simulink model "SLX_HoqueSimulink"  (R2025a)
settings: Solver=VariableStepAuto  StartTime=0.0  StopTime=inf  RelTol=1e-3
values from neighbouring files (symbols this model uses):
  Cd = 0.5    [SLX_HoqueMatlab.m]
  centreOfMassHeight = 0.5    [SLX_HoqueMatlab.m]
  frontExposedArea = 0.3    [SLX_HoqueMatlab.m]
  g = 9.81    [SLX_HoqueMatlab.m]
  inertia = 1    [SLX_HoqueMatlab.m]
  mass = 200    [SLX_HoqueMatlab.m]
  radius = 0.3    [SLX_HoqueMatlab.m]
  rhoAir = 1.225    [SLX_HoqueMatlab.m]
  wheelbase = 1.4    [SLX_HoqueMatlab.m]
libraries: slpidlib x2
settings Model: PacingRate=0.710000  Creator=rafiu  LastModifiedBy=rafiu

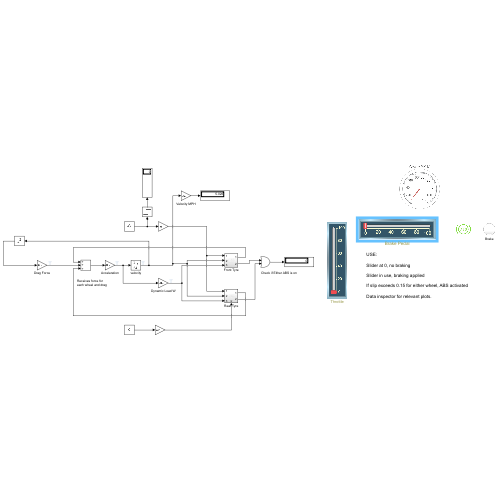
[thumbnail: Simulink's stored preview of the top-level diagram]
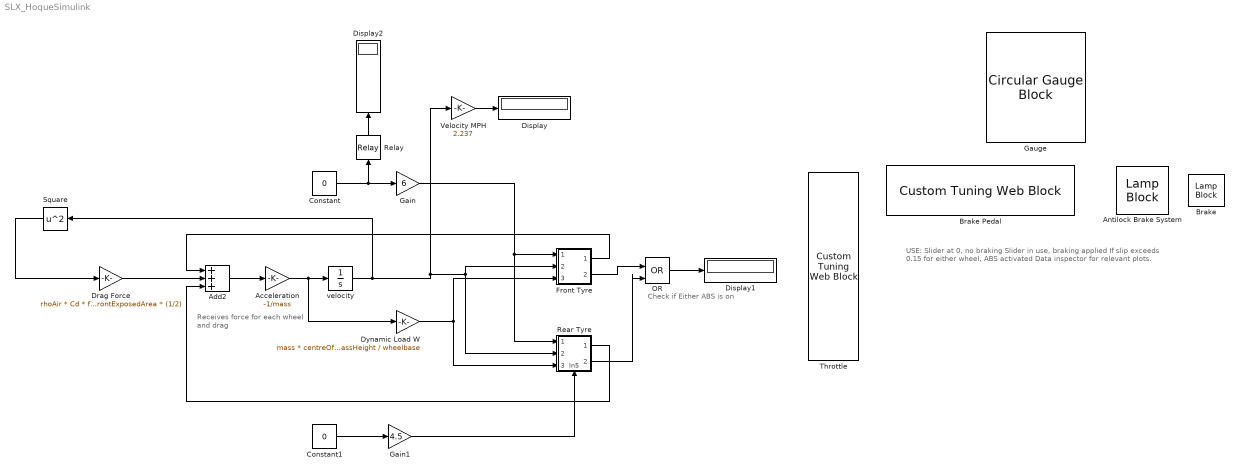
== system SLX_HoqueSimulink ==
  note: Receives force for each wheel and drag
  note: Check if Either ABS is on
  note: USE:
      |
      | Slider at 0, no braking
      |
      | Slider in use, braking applied
      |
      | If slip exceeds 0.15 for either wheel, ABS activated
      |
      | Data inspector for relevant plots.
  Acceleration : Gain  Gain=-1/mass
  Add2 : Sum  Inputs=+++
  Antilock Brake System : LampBlock  LabelPosition=Hide  DefaultColor=[192.0, 192.0, 192.0]  Icon=AntilockBrakeSystem
  Brake : LampBlock  LabelPosition=Hide  DefaultColor=[192.0, 192.0, 192.0]
  Brake Pedal : CustomTuningWebBlock  LabelPosition=Hide  ShowInitialText=on  Configuration="{\"components\":[{\"name\":\"LinearScaleComponent\",\"settings\":{\"bounds\":{\"max\":100,\"min\":0,\"tickInterval\":\"auto\"},\"internalTickHeightScaleFactor\":0.5,\"labelColor\":[255,255,200],\"labelFont\":{\"font\":\"Arial\",\"fontSize\":12},\"labelOffset\":0.05,\"labelTransparency\":1,\"needleImage\":{\"size\":[596,842],\"src\":\"data:image\\/svg+xml;base64,PD94bWwgdmVyc2lvbj0iMS4wIiBlbmNvZGluZz0idXRmLTgiPz4NCjwhLS0gR2VuZXJhdG9yOiBBZG9iZSBJbGx1c3RyYXRvciAyNS4wLjAsIFNWRyBFeHBvcnQgUGx1Zy1JbiAuIFNWRyBWZXJzaW9uOiA2LjAwIEJ1aWxkIDApICAtLT4NCjxzdmcgdmVyc2lvbj0iMS4xIg0KCSBpZD0ic3ZnOCIgeG1sbnM6Y2M9Imh0dHA6Ly9jcmVhdGl2ZWNvbW1vbnMub3JnL25zIyIgeG1sbnM6ZGM9Imh0dHA6Ly9wdXJsLm9yZy9kYy9lbGVtZW50cy8xLjEvIiB4bWxuczppbmtzY2FwZT0iaHR0cDovL3d3dy5pbmtzY2FwZS5vcmcvbmFtZXNw ...(+2420 chars)\",\"srcOrientation\":\"Right\"},\"needleOffset\":[-0.8044596912521441,-0.0642123287671233],\"needleSize\":{\"height\":0.4337797619047619,\"width\":0.07668067226890757},\"position\":[0.2829861111111111,0.04398634453781513,0.9196428571428571,0.6088789682539683],\"referencePoint\":\"auto\",\"scaleColors\":[],\"scaleColorsSize\":0.2,\"scaleDirection\":\"LR\",\"showLabels\":1,\"showMinorTicks\":0,\"showSpanLine\":1,\"showTicks\":1,\"tickColor\":[252,252,197],\"tickTransparency\":1,\"valueBarColor\":[0,114,189],\"valueBarOffset\":-0.27,\"valueBarSize\":0.1,\"valueBarTransparency\":1}},{\"name\":\"BackgroundImageComponent\",\"settings\":{\"image\":{\"size\":[380,101],\"src\":\"data:image\\/svg+xml;base64,PHN2ZyB4bWxucz0iaHR0cDovL3d3dy53My5vcmcvMjAwMC9zdmciIHhtbG5zOnhsaW5rPSJodHRwOi8vd3d3LnczLm9yZy8xOTk5L3hsaW5rIiB2aWV3Qm94PSIwIDAgMzgwIDEwMSI+PGRlZnM+PHN0eWxlPi5jbHMtMXtmaWxsOiMwMDJiNDI7fS5jbHMtMntmaWxsOiM0MjcwODI7fS5jbHMtM3tmaWxsOnVybCgjcmFkaWFsLWdyYWRpZW50KTt9LmNscy00e2ZpbGw6I2M4YzhjODtzdHJva2U6IzAwMDt9PC9zdHlsZT48cmFkaWFsR3JhZGllbnQgaWQ9InJhZGlhbC1ncmFkaWVudCIgY3g9IjE5MCIgY3k9IjUwLjUiIHI9IjI2OS4yMSIgZ3JhZGllbnRVbml0cz0idXNlclNwYWNlT25Vc2UiPjxzdG9wIG9mZnNldD0iMC4wMSIgc3RvcC1jb2xvcj0iIzNlNGY1OCIvPjxzdG9wIG9mZnNldD0iMC4wNiIgc3RvcC1jb2xvcj0iIzQ0NTc2MSIvPjxzdG9wIG9mZnNldD0iMC4xNSIgc3RvcC1jb2xvcj0iIzU1NmE3NiIvPjxzdG9wIG9mZnNldD0iMC4yNSIgc3RvcC1jb2xvcj0iIzZkODg5NSIvPjxzdG9wIG9mZnNldD0iMC4zOCIgc3RvcC1jb2xvcj0iIzhmYjJjMyIvPjxzdG9wIG9mZnNldD0iMC41MiIgc3RvcC1jb2xvcj0iI2I2ZTRmYSIvPjxzdG9wIG9mZnNldD0iMSIgc3RvcC1jb2xvcj0iIzE1NDY1NyIvPjwvcmFkaWFsR3JhZGllbnQ+PC9kZWZzPjxnIGlkPSJmcmFtZSI+PGcgaWQ9IkxheWVyXzIiIGRhdGEtbmFtZT0iTGF5ZXIgMiI+PGcgaWQ9IkxheWVyXzEtMiIgZGF0YS1uYW1lPSJMYXllciAxLTIiPjxyZWN0IGlkPSJyZWN0MTAzNiIgY2xhc3M9ImNscy0xIiB4PSIxMSIgeT0iMTEiIHdpZHRoPSIzNTgiIGhlaWdodD0iNzkiLz48cGF0aCBpZD0icGF0aDEwMzgiIGNsYXNzPSJjbHMtMiIgZD0iTTgsOFY5M0gzNzJWOFpNMzY5LDkwSDExVjExSDM2OVoiLz48cGF0aCBpZD0icGF0aDEwNDAiIGNsYXNzPSJjbHMtMyIgZD0iTTAsMFYxMDFIMzgwVjBaTTM3Miw5M0g4VjhIMzcyWiIvPjwvZz48L2c+PC9nPjxnIGlkPSJ0cmFjayI+PHBhdGggaWQ9InJlY3QxNjExIiBjbGFzcz0iY2xzLTQiIGQ9Ik0zMy4zNywyNi41OUgzNDYuNjNjNCwwLDcuMjUsMi42LDcuMjUsNS44MWgwYzAsMy4yMS0zLjI1LDUuODItNy4yNSw1LjgySDMzLjM3Yy00LDAtNy4yNS0yLjYxLTcuMjUtNS44MmgwQzI2LjEyLDI5LjE5LDI5LjM3LDI2LjU5LDMzLjM3LDI2LjU5WiIvPjwvZz48L3N2Zz4=\",\"srcOrientation\":\"horizontal\"},\"position\":[0,0,1,1],\"scaleMode\":\"0\"}},{\"name\":\"ForegroundImageComponent\",\"settings\":{\"image\":{\"size\":[0,0],\"src\":\"default\",\"srcOrientation\":[]},\"isForeground\":1,\"position\":[0,0,1,1],\"scaleMode\":\"0\"}}],\"derived\":{\"blockParameters\":{\"ForegroundColor\":[0.9882352941176471,0.9882352941176471,0.7725490196078432],\"Limits\":{\"Max\":100,\"Min\":0,\"Ticks\":\"auto\"},\"ScaleColors\":[],\"ScaleDirection\":\"Clockwise\",\"ScaleMax\":100,\"ScaleMin\":0,\"TickInterval\":\"auto\",\"fixedAspectRatio\":\"on\"}},\"settings\":{\"BindingType\":\"param\",\"aspectRatio\":3.7777777777777777,\"backgroundColor\":[0,0,0,\"1\"],\"backgroundOffset\":0,\"backgroundOpacity\":1,\"fixedAspectRatio\":\"on\",\"foregroundColor\":[252,252,196],\"orientation\":\"horizontal\",\"showBackgroundColor\":false,\"value\":0,\"version\":\"R2023a\"},\"type\":\"LinearGauge\"}"
  Constant : Constant  Value=0
  Constant1 : Constant  Value=0
  Display : Display
  Display1 : Display
  Display2 : Display
  Drag Force : Gain  Gain=rhoAir * Cd * frontExposedArea * (1/2)
  Dynamic Load W : Gain  Gain=mass * centreOfMassHeight / wheelbase
  Front Tyre : Subsystem
  Gain : Gain  Gain=6
  Gain1 : Gain  Gain=4.5
  Gauge : CircularGaugeBlock  ScaleMax=180  FontColor=[0.0, 0.0, 0.0]
  OR : Logic  Operator=OR  IconShape=distinctive  AllPortsSameDT=off  OutDataTypeStr=boolean
  Rear Tyre : Subsystem
      settings: PortSchema="{\"entries\":[{\"content\":{\"sides\":[{\"content\":{\"connectorIds\":[\"In1\",\"In2\",\"In3\"]},\"type\":\"ConnectorPlacement.EquallySpacedRectSide\",\"uuid\":\"1266f35d-f5b4-4b9c-be11-d6befbdb1413\"},{\"content\":{\"connectorIds\":[\"Out1\",\"Out2\"],\"side\":\"RIGHT\"},\"type\":\"ConnectorPlacement.EquallySpacedRectSide\",\"uuid\":\"caeb7587-b63b-4911-94e2-b6cf9e0b40d6\"},{\"content\":{\"side\":\"TOP\"},\"type\":\"ConnectorPlacement.EquallySpacedRectSide\",\"uuid\":\"79f45d0a-d588-4f96-966e-94542620e09c\"},{\"content\":{\"connectorIds\":[\"In4\"],\"side\":\"BOTTOM\"},\"type\":\"ConnectorPlacement.EquallySpacedRectSide\",\"uuid\":\"f75c0003-57c9-4cd0-88eb-cf91023de0b2\"}]},\"type\":\"ConnectorPlacement.EquallySpacedConnector\",\"uuid\":\"6a6eede2-c9ff-4d9d-a3d1-7dc9cb2ac1d3\"}],\"packageUris\":[\"http://schema.mathworks.com/mf0/Connector/R2020b\"],\"version\":\"1.0\"}"
  Relay : Relay  OnSwitchValue=0.1  OffSwitchValue=0
  Square : Math  Operator=square
  Throttle : CustomTuningWebBlock  LabelPosition=Hide  ShowInitialText=on  Configuration="{\"components\":[{\"name\":\"LinearScaleComponent\",\"settings\":{\"bounds\":{\"max\":100,\"min\":0,\"tickInterval\":\"auto\"},\"internalTickHeightScaleFactor\":0.5,\"labelColor\":[255,255,200],\"labelFont\":{\"font\":\"Arial\",\"fontSize\":12},\"labelOffset\":0.05,\"labelTransparency\":1,\"needleImage\":{\"size\":[596,842],\"src\":\"data:image\\/svg+xml;base64,PD94bWwgdmVyc2lvbj0iMS4wIiBlbmNvZGluZz0idXRmLTgiPz4NCjwhLS0gR2VuZXJhdG9yOiBBZG9iZSBJbGx1c3RyYXRvciAyNS4wLjAsIFNWRyBFeHBvcnQgUGx1Zy1JbiAuIFNWRyBWZXJzaW9uOiA2LjAwIEJ1aWxkIDApICAtLT4NCjxzdmcgdmVyc2lvbj0iMS4xIg0KCSBpZD0ic3ZnOCIgeG1sbnM6Y2M9Imh0dHA6Ly9jcmVhdGl2ZWNvbW1vbnMub3JnL25zIyIgeG1sbnM6ZGM9Imh0dHA6Ly9wdXJsLm9yZy9kYy9lbGVtZW50cy8xLjEvIiB4bWxuczppbmtzY2FwZT0iaHR0cDovL3d3dy5pbmtzY2FwZS5vcmcvbmFtZXNw ...(+2420 chars)\",\"srcOrientation\":\"horizontal\"},\"needleOffset\":[0.0642123287671233,-0.8044596912521441],\"needleSize\":{\"height\":0.07668067226890757,\"width\":0.4337797619047619},\"position\":[0.03623949579831933,0.2829861111111111,0.6088789682539683,0.9196428571428571],\"referencePoint\":\"auto\",\"scaleColors\":[],\"scaleColorsSize\":0.2,\"scaleDirection\":\"BT\",\"showLabels\":1,\"showMinorTicks\":0,\"showSpanLine\":1,\"showTicks\":1,\"tickColor\":[252,252,197],\"tickTransparency\":1,\"valueBarColor\":[0,114,189],\"valueBarOffset\":-0.27,\"valueBarSize\":0.1,\"valueBarTransparency\":1}},{\"name\":\"BackgroundImageComponent\",\"settings\":{\"image\":{\"size\":[380,101],\"src\":\"data:image\\/svg+xml;base64,PHN2ZyB4bWxucz0iaHR0cDovL3d3dy53My5vcmcvMjAwMC9zdmciIHhtbG5zOnhsaW5rPSJodHRwOi8vd3d3LnczLm9yZy8xOTk5L3hsaW5rIiB2aWV3Qm94PSIwIDAgMzgwIDEwMSI+PGRlZnM+PHN0eWxlPi5jbHMtMXtmaWxsOiMwMDJiNDI7fS5jbHMtMntmaWxsOiM0MjcwODI7fS5jbHMtM3tmaWxsOnVybCgjcmFkaWFsLWdyYWRpZW50KTt9LmNscy00e2ZpbGw6I2M4YzhjODtzdHJva2U6IzAwMDt9PC9zdHlsZT48cmFkaWFsR3JhZGllbnQgaWQ9InJhZGlhbC1ncmFkaWVudCIgY3g9IjE5MCIgY3k9IjUwLjUiIHI9IjI2OS4yMSIgZ3JhZGllbnRVbml0cz0idXNlclNwYWNlT25Vc2UiPjxzdG9wIG9mZnNldD0iMC4wMSIgc3RvcC1jb2xvcj0iIzNlNGY1OCIvPjxzdG9wIG9mZnNldD0iMC4wNiIgc3RvcC1jb2xvcj0iIzQ0NTc2MSIvPjxzdG9wIG9mZnNldD0iMC4xNSIgc3RvcC1jb2xvcj0iIzU1NmE3NiIvPjxzdG9wIG9mZnNldD0iMC4yNSIgc3RvcC1jb2xvcj0iIzZkODg5NSIvPjxzdG9wIG9mZnNldD0iMC4zOCIgc3RvcC1jb2xvcj0iIzhmYjJjMyIvPjxzdG9wIG9mZnNldD0iMC41MiIgc3RvcC1jb2xvcj0iI2I2ZTRmYSIvPjxzdG9wIG9mZnNldD0iMSIgc3RvcC1jb2xvcj0iIzE1NDY1NyIvPjwvcmFkaWFsR3JhZGllbnQ+PC9kZWZzPjxnIGlkPSJmcmFtZSI+PGcgaWQ9IkxheWVyXzIiIGRhdGEtbmFtZT0iTGF5ZXIgMiI+PGcgaWQ9IkxheWVyXzEtMiIgZGF0YS1uYW1lPSJMYXllciAxLTIiPjxyZWN0IGlkPSJyZWN0MTAzNiIgY2xhc3M9ImNscy0xIiB4PSIxMSIgeT0iMTEiIHdpZHRoPSIzNTgiIGhlaWdodD0iNzkiLz48cGF0aCBpZD0icGF0aDEwMzgiIGNsYXNzPSJjbHMtMiIgZD0iTTgsOFY5M0gzNzJWOFpNMzY5LDkwSDExVjExSDM2OVoiLz48cGF0aCBpZD0icGF0aDEwNDAiIGNsYXNzPSJjbHMtMyIgZD0iTTAsMFYxMDFIMzgwVjBaTTM3Miw5M0g4VjhIMzcyWiIvPjwvZz48L2c+PC9nPjxnIGlkPSJ0cmFjayI+PHBhdGggaWQ9InJlY3QxNjExIiBjbGFzcz0iY2xzLTQiIGQ9Ik0zMy4zNywyNi41OUgzNDYuNjNjNCwwLDcuMjUsMi42LDcuMjUsNS44MWgwYzAsMy4yMS0zLjI1LDUuODItNy4yNSw1LjgySDMzLjM3Yy00LDAtNy4yNS0yLjYxLTcuMjUtNS44MmgwQzI2LjEyLDI5LjE5LDI5LjM3LDI2LjU5LDMzLjM3LDI2LjU5WiIvPjwvZz48L3N2Zz4=\",\"srcOrientation\":\"horizontal\"},\"position\":[0,0,1,1],\"scaleMode\":\"0\"}},{\"name\":\"ForegroundImageComponent\",\"settings\":{\"image\":{\"size\":[0,0],\"src\":\"default\",\"srcOrientation\":[]},\"isForeground\":1,\"position\":[0,0,1,1],\"scaleMode\":\"0\"}}],\"derived\":{\"blockParameters\":{\"ForegroundColor\":[0.9882352941176471,0.9882352941176471,0.7725490196078432],\"Limits\":{\"Max\":100,\"Min\":0,\"Ticks\":\"auto\"},\"ScaleColors\":[],\"ScaleDirection\":\"Clockwise\",\"ScaleMax\":100,\"ScaleMin\":0,\"TickInterval\":\"auto\",\"fixedAspectRatio\":\"on\"}},\"settings\":{\"BindingType\":\"param\",\"aspectRatio\":3.7777777777777777,\"backgroundColor\":[0,0,0,\"1\"],\"backgroundOffset\":0,\"backgroundOpacity\":1,\"fixedAspectRatio\":\"on\",\"foregroundColor\":[252,252,196],\"orientation\":\"vertical\",\"showBackgroundColor\":false,\"value\":0,\"version\":\"R2023a\"},\"type\":\"LinearGauge\"}"
  Velocity MPH : Gain  Gain=2.237
  velocity : Integrator  InitialCondition=25  LimitOutput=on  LowerSaturationLimit=0.1
  wires:
  Acceleration/1 -> Dynamic Load W/1, velocity/1
  Add2/1 -> Acceleration/1
  Dynamic Load W/1 -> Rear Tyre/3(In2), Front Tyre/3(In2)
  Front Tyre/1(Out1) -> Add2/1
  Constant/1 -> Gain/1, Relay/1
  Gain/1 -> Front Tyre/1(1), Rear Tyre/1(In3)
  Velocity MPH/1 -> Display/1
  OR/1 -> Display1/1
  Front Tyre/2(Out2) -> OR/1
  Rear Tyre/2(Out2) -> OR/2
  Relay/1 -> Display2/1
  Constant1/1 -> Gain1/1
  Gain1/1 -> Rear Tyre/4(In5)
  velocity/1 -> Square/1, Velocity MPH/1, Front Tyre/2(In1), Rear Tyre/2(In1)
  Rear Tyre/1(Out1) -> Add2/3
  Square/1 -> Drag Force/1
  Drag Force/1 -> Add2/2

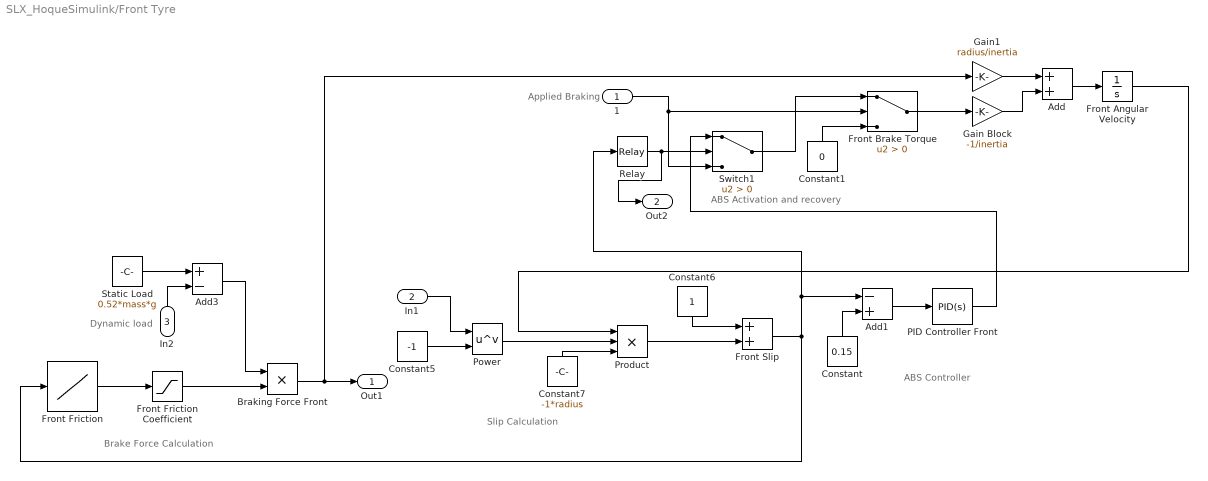
== system SLX_HoqueSimulink/Front Tyre ==
  note: Dynamic load
  note: Brake Force Calculation
  note: ABS Activation and recovery
  note: Applied Braking
  note: Slip Calculation
  note: ABS Controller
  1 : Inport
  In1 : Inport  Port=2
  In2 : Inport  Port=3
  Add : Sum
  Add1 : Sum  Inputs=-+
  Add3 : Sum  Inputs=+-
  Braking Force Front : Product
  Constant : Constant  Value=0.15
  Constant1 : Constant  Value=0
  Constant5 : Constant  Value=-1
  Constant6 : Constant
  Constant7 : Constant  Value=-1*radius
  "Front Angular Velocity " : Integrator  InitialCondition=83.33  LimitOutput=on  LowerSaturationLimit=0
  Front Brake Torque : Switch  Criteria=u2 > Threshold  SaturateOnIntegerOverflow=off  InputSameDT=off
  Front Friction : Lookup_n-D  NumberOfTableDimensions=1  BreakpointsForDimension1=[-1;-0.5;-0.29999999999999999;-0.20000000000000001;-0.14999999999999999;-0.10000000000000001;-0.050000000000000003;0;0.050000000000000003;0.10000000000000001;0.14999999999999999;0.20000000000000001;0.29999999999999999;0.5;1]  Table=[-0.10000000000000001;-0.40000000000000002;-0.75;-0.94999999999999996;-1;-0.90000000000000002;-0.59999999999999998;0;0.59999999999999998;0.90000000000000002;1;0.94999999999999996;0.75;0.40000000000000002;0.10000000000000001]  InternalRulePriority=Speed  RndMeth=Simplest
  Front Friction Coefficient : Saturate  UpperLimit=1  LowerLimit=-1
  Front Slip : Sum
  Gain Block : Gain  Gain=-1/inertia
  Gain1 : Gain  Gain=radius/inertia
  PID Controller Front : slpidlib/PID Controller  Controller=PID  Form=Parallel  TimeDomain=Continuous-time  UseExternalTs=off  SampleTime=-1  IntegratorMethod=Forward Euler  FilterMethod=Forward Euler  ControllerParametersSource=internal  P=6397.12321645697  I=564779.033744015  UseKiTs=off  D=-9.50321064069282  UseExternalDerivativeSource=off  N=94.2884376417399  UseFilter=on  TunerSelectOption=Transfer Function Based (PID Tuner App)  InitialConditionSource=internal  InitialConditionForIntegrator=0  InitialConditionForFilter=0  DifferentiatorICPrevScaledInput=0  ExternalReset=none  TrackingMode=off  Kt=1  LimitOutput=on  SatLimitsSource=internal  UpperSaturationLimit=600  LowerSaturationLimit=0  LinearizeAsGain=on  AntiWindupMode=back-calculation  Kb=1  LimitIntegrator=on  UpperIntegratorSaturationLimit=1000  LowerIntegratorSaturationLimit=-inf  POutMin=[]  POutMax=[]  IOutMin=[]  IOutMax=[]  DOutMin=[]  DOutMax=[]  NOutMin=[]  NOutMax=[]  SumOutMin=[]  SumOutMax=[]  SaturationOutMin=[]  SaturationOutMax=[]  PParamMin=[]  PParamMax=[]  IParamMin=[]  IParamMax=[]  DParamMin=[]  DParamMax=[]  NParamMin=[]  NParamMax=[]  KbParamMin=[]  KbParamMax=[]  KtParamMin=[]  KtParamMax=[]  KbOutMin=[]  KbOutMax=[]  KtOutMin=[]  KtOutMax=[]  IntegratorOutMin=[]  IntegratorOutMax=[]  FilterOutMin=[]  FilterOutMax=[]  SumI1OutMin=[]  SumI1OutMax=[]  SumI2OutMin=[]  SumI2OutMax=[]  SumI3OutMin=[]  SumI3OutMax=[]  SumI4OutMin=[]  SumI4OutMax=[]  SumDOutMin=[]  SumDOutMax=[]  DifferentiatorOutMin=[]  DifferentiatorOutMax=[]  FilterDiffOutCoefMin=[]  FilterDiffOutCoefMax=[]  ReciprocalOutMin=[]  ReciprocalOutMax=[]  SumDenOutMin=[]  SumDenOutMax=[]  SumNumOutMin=[]  SumNumOutMax=[]  DivideOutMin=[]  DivideOutMax=[]  UdiffTsProdOutMin=[]  UdiffTsProdOutMax=[]  NTsProdOutMin=[]  NTsProdOutMax=[]  UintegralTsProdOutMin=[]  UintegralTsProdOutMax=[]  UngainTsProdOutMin=[]  UngainTsProdOutMax=[]  ClampingZeroOutDataTypeStr=Inherit: Inherit via back propagation  ClampingZeroOutMin=[]  ClampingZeroOutMax=[]  FilterDenConstantOutDataTypeStr=Inherit: Inherit via back propagation  FilterDenConstantOutMin=[]  FilterDenConstantOutMax=[]  PCopyOutDataTypeStr=Inherit: Inherit via back propagation  PCopyOutMin=[]  PCopyOutMax=[]  NCopyOutDataTypeStr=Inherit: Inherit via back propagation  NCopyOutMin=[]  NCopyOutMax=[]  IntegratorContinuousStateAttributes=''  IntegratorStateMustResolveToSignalObject=off  IntegratorRTWStateStorageClass=Auto  FilterContinuousStateAttributes=''  FilterStateMustResolveToSignalObject=off  FilterRTWStateStorageClass=Auto  ParallelPVariant=InternalParameters  IdealPVariant=Disabled  IVariant=InternalParameters  DVariant=InternalParameters  IntegratorVariant=Continuous  SatVariant=Enabled  AWVariant=BackCalculation  PCopyVariant=Disabled  TRVariant=Disabled  FdbkBlocksVariant=Forward  IdealPFdbkVariant=Disabled  SatFdbkVariant=Disabled  DerivativeFilterVariant=ContFilter  NVariant=InternalParameters  NCopyVariant=Disabled  FilterICVariant=InternalICsFilter  IntegratorICVariant=InternalICs  ExternalResetVariant=Disabled  TRSumVariant=Passthrough  SumFdbkVariant=Disabled  SumVariant=Sum_PID  TsampFilterVariant=InternalTs  TsampNgainVariant=Passthrough  TsampIntegralVariant=Disabled_SignalSpec  ExternalSaturationOutDataTypeStr=Inherit: Same as second input  DerivativeSourceVariant=ErrorSignal  PreIntVariant=InternalPreInt
  Power : Math  Operator=pow
  Product : Product  Inputs=3
  Relay : Relay  OnSwitchValue=0.15  OffSwitchValue=0.1
  Static Load : Constant  Value=0.52*mass*g
  Switch1 : Switch  Criteria=u2 > Threshold  SaturateOnIntegerOverflow=off  InputSameDT=off
  Out1 : Outport
  Out2 : Outport  Port=2
  wires:
  Front Slip/1 -> Front Friction/1, Relay/1, Add1/1
  "Front Angular Velocity "/1 -> Product/1
  Gain1/1 -> Add/1
  Constant6/1 -> Front Slip/1
  Product/1 -> Front Slip/2
  Gain Block/1 -> Add/2
  Constant5/1 -> Power/2
  Add/1 -> "Front Angular Velocity "/1
  Constant7/1 -> Product/3
  Braking Force Front/1 -> Out1/1, Gain1/1
  Power/1 -> Product/2
  Front Friction/1 -> Front Friction Coefficient/1
  Static Load/1 -> Add3/1
  Add3/1 -> Braking Force Front/1
  In2/1 -> Add3/2
  In1/1 -> Power/1
  Front Friction Coefficient/1 -> Braking Force Front/2
  Constant/1 -> Add1/2
  Add1/1 -> PID Controller Front/1
  1/1 -> Switch1/3, Front Brake Torque/2
  Switch1/1 -> Front Brake Torque/1
  Constant1/1 -> Front Brake Torque/3
  Relay/1 -> Out2/1, Switch1/2
  PID Controller Front/1 -> Switch1/1
  Front Brake Torque/1 -> Gain Block/1

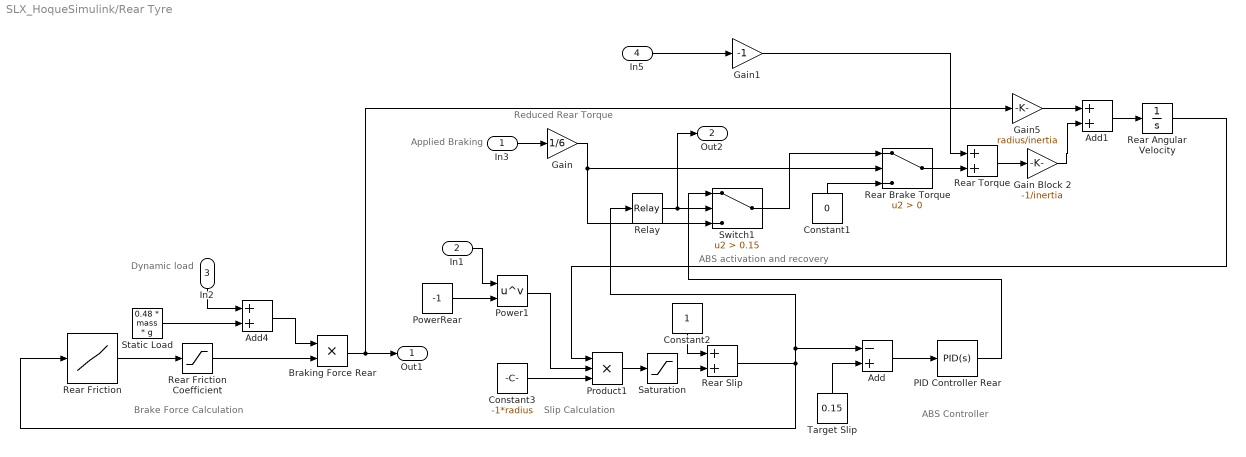
== system SLX_HoqueSimulink/Rear Tyre ==
  note: Dynamic load
  note: Reduced Rear Torque
  note: Applied Braking
  note: Brake Force Calculation
  note: Slip Calculation
  note: ABS Controller
  note: ABS activation and recovery
  In3 : Inport
  In1 : Inport  Port=2
  In2 : Inport  Port=3
  In5 : Inport  Port=4
  Add : Sum  Inputs=-+
  Add1 : Sum
  Add4 : Sum
  Braking Force Rear : Product
  Constant1 : Constant  Value=0
  Constant2 : Constant
  Constant3 : Constant  Value=-1*radius
  Gain : Gain  Gain=1/6
  Gain Block 2 : Gain  Gain=-1/inertia
  Gain1 : Gain  Gain=-1
  Gain5 : Gain  Gain=radius/inertia
  PID Controller Rear : slpidlib/PID Controller  Controller=PID  Form=Parallel  TimeDomain=Continuous-time  UseExternalTs=off  SampleTime=-1  IntegratorMethod=Forward Euler  FilterMethod=Forward Euler  ControllerParametersSource=internal  P=63649.2747013597  I=14488550.6252492  UseKiTs=off  D=-7.50563341365421  UseExternalDerivativeSource=off  N=8480.20029669571  UseFilter=on  TunerSelectOption=Transfer Function Based (PID Tuner App)  InitialConditionSource=internal  InitialConditionForIntegrator=0  InitialConditionForFilter=0  DifferentiatorICPrevScaledInput=0  ExternalReset=none  TrackingMode=off  Kt=1  LimitOutput=on  SatLimitsSource=internal  UpperSaturationLimit=100  LowerSaturationLimit=0  LinearizeAsGain=on  AntiWindupMode=back-calculation  Kb=1  LimitIntegrator=on  UpperIntegratorSaturationLimit=1000  LowerIntegratorSaturationLimit=-inf  POutMin=[]  POutMax=[]  IOutMin=[]  IOutMax=[]  DOutMin=[]  DOutMax=[]  NOutMin=[]  NOutMax=[]  SumOutMin=[]  SumOutMax=[]  SaturationOutMin=[]  SaturationOutMax=[]  PParamMin=[]  PParamMax=[]  IParamMin=[]  IParamMax=[]  DParamMin=[]  DParamMax=[]  NParamMin=[]  NParamMax=[]  KbParamMin=[]  KbParamMax=[]  KtParamMin=[]  KtParamMax=[]  KbOutMin=[]  KbOutMax=[]  KtOutMin=[]  KtOutMax=[]  IntegratorOutMin=[]  IntegratorOutMax=[]  FilterOutMin=[]  FilterOutMax=[]  SumI1OutMin=[]  SumI1OutMax=[]  SumI2OutMin=[]  SumI2OutMax=[]  SumI3OutMin=[]  SumI3OutMax=[]  SumI4OutMin=[]  SumI4OutMax=[]  SumDOutMin=[]  SumDOutMax=[]  DifferentiatorOutMin=[]  DifferentiatorOutMax=[]  FilterDiffOutCoefMin=[]  FilterDiffOutCoefMax=[]  ReciprocalOutMin=[]  ReciprocalOutMax=[]  SumDenOutMin=[]  SumDenOutMax=[]  SumNumOutMin=[]  SumNumOutMax=[]  DivideOutMin=[]  DivideOutMax=[]  UdiffTsProdOutMin=[]  UdiffTsProdOutMax=[]  NTsProdOutMin=[]  NTsProdOutMax=[]  UintegralTsProdOutMin=[]  UintegralTsProdOutMax=[]  UngainTsProdOutMin=[]  UngainTsProdOutMax=[]  ClampingZeroOutDataTypeStr=Inherit: Inherit via back propagation  ClampingZeroOutMin=[]  ClampingZeroOutMax=[]  FilterDenConstantOutDataTypeStr=Inherit: Inherit via back propagation  FilterDenConstantOutMin=[]  FilterDenConstantOutMax=[]  PCopyOutDataTypeStr=Inherit: Inherit via back propagation  PCopyOutMin=[]  PCopyOutMax=[]  NCopyOutDataTypeStr=Inherit: Inherit via back propagation  NCopyOutMin=[]  NCopyOutMax=[]  IntegratorContinuousStateAttributes=''  IntegratorStateMustResolveToSignalObject=off  IntegratorRTWStateStorageClass=Auto  FilterContinuousStateAttributes=''  FilterStateMustResolveToSignalObject=off  FilterRTWStateStorageClass=Auto  ParallelPVariant=InternalParameters  IdealPVariant=Disabled  IVariant=InternalParameters  DVariant=InternalParameters  IntegratorVariant=Continuous  SatVariant=Enabled  AWVariant=BackCalculation  PCopyVariant=Disabled  TRVariant=Disabled  FdbkBlocksVariant=Forward  IdealPFdbkVariant=Disabled  SatFdbkVariant=Disabled  DerivativeFilterVariant=ContFilter  NVariant=InternalParameters  NCopyVariant=Disabled  FilterICVariant=InternalICsFilter  IntegratorICVariant=InternalICs  ExternalResetVariant=Disabled  TRSumVariant=Passthrough  SumFdbkVariant=Disabled  SumVariant=Sum_PID  TsampFilterVariant=InternalTs  TsampNgainVariant=Passthrough  TsampIntegralVariant=Disabled_SignalSpec  ExternalSaturationOutDataTypeStr=Inherit: Same as second input  DerivativeSourceVariant=ErrorSignal  PreIntVariant=InternalPreInt
  Power1 : Math  Operator=pow
  PowerRear : Constant  Value=-1
  Product1 : Product  Inputs=3
  Rear Angular Velocity : Integrator  InitialCondition=83.33  LimitOutput=on  UpperSaturationLimit=80/radius  LowerSaturationLimit=0
  Rear Brake Torque : Switch  Criteria=u2 > Threshold  SaturateOnIntegerOverflow=off  InputSameDT=off
  Rear Friction : Lookup_n-D  NumberOfTableDimensions=1  BreakpointsForDimension1=[-1;-0.5;-0.29999999999999999;-0.20000000000000001;-0.14999999999999999;-0.10000000000000001;-0.050000000000000003;0;0.050000000000000003;0.10000000000000001;0.14999999999999999;0.20000000000000001;0.29999999999999999;0.5;1]  Table=[-0.10000000000000001;-0.40000000000000002;-0.75;-0.94999999999999996;-1;-0.90000000000000002;-0.59999999999999998;0;0.59999999999999998;0.90000000000000002;1;0.94999999999999996;0.75;0.40000000000000002;0.10000000000000001]  InternalRulePriority=Speed  RndMeth=Simplest
  Rear Friction Coefficient : Saturate  UpperLimit=1  LowerLimit=-1
  Rear Slip : Sum
  Rear Torque : Sum
  Relay : Relay  OnSwitchValue=0.15  OffSwitchValue=0.1
  Saturation : Saturate  UpperLimit=-0.01  LowerLimit=-1.99
  Static Load : Constant  Value=0.48 * mass * g
  Switch1 : Switch  Criteria=u2 > Threshold  Threshold=0.15  SaturateOnIntegerOverflow=off  InputSameDT=off
  Target Slip : Constant  Value=0.15
  Out1 : Outport
  Out2 : Outport  Port=2
  wires:
  Rear Friction/1 -> Rear Friction Coefficient/1
  PowerRear/1 -> Power1/2
  Rear Friction Coefficient/1 -> Braking Force Rear/2
  Braking Force Rear/1 -> Out1/1, Gain5/1
  Rear Angular Velocity/1 -> Product1/1
  Power1/1 -> Product1/2
  Constant3/1 -> Product1/3
  Static Load/1 -> Add4/2
  In1/1 -> Power1/1
  Constant2/1 -> Rear Slip/1
  Gain Block 2/1 -> Add1/2
  In2/1 -> Add4/1
  Product1/1 -> Saturation/1
  Add1/1 -> Rear Angular Velocity/1
  Gain5/1 -> Add1/1
  Add4/1 -> Braking Force Rear/1
  Target Slip/1 -> Add/2
  Add/1 -> PID Controller Rear/1
  In3/1 -> Gain/1
  Constant1/1 -> Rear Brake Torque/3
  Switch1/1 -> Rear Brake Torque/1
  Relay/1 -> Out2/1, Switch1/2
  Gain/1 -> Switch1/3, Rear Brake Torque/2
  PID Controller Rear/1 -> Switch1/1
  Rear Brake Torque/1 -> Rear Torque/2
  Rear Torque/1 -> Gain Block 2/1
  Gain1/1 -> Rear Torque/1
  In5/1 -> Gain1/1
  Rear Slip/1 -> Relay/1, Add/1, Rear Friction/1
  Saturation/1 -> Rear Slip/2
